simulink model "udp_scenario"  (R2024b)
settings: Solver=FixedStepDiscrete  StartTime=0.0  StopTime=90  RelTol=1e-3
model workspace (MAT data in the model file):
  firstWarning = 1
  originalScenarioChecksum = 'E10BFE42C1659D1EFEE8B4DF190BE309'
libraries: drivingscenarioandsensors x1
settings Model: Creator=jheitmann  LastModifiedBy=jheitmann

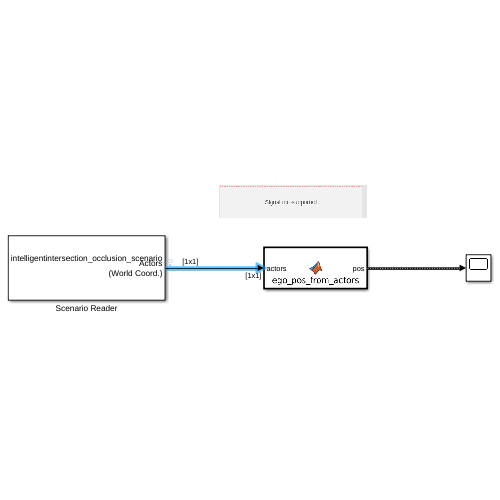
[thumbnail: Simulink's stored preview of the top-level diagram]
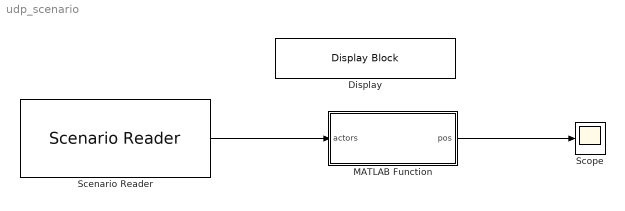
== system udp_scenario ==
  Display : DisplayBlock  LabelPosition=Hide  Transparency=1
  MATLAB Function : MATLAB Function  TreatAsAtomicUnit=on
  Scenario Reader : drivingscenarioandsensors/Scenario Reader  ScenarioSource=From file  ScenarioFileName=/home/jheitmann/MATLAB/Projects/intintersection/intelligentintersection_occlusion_scenario.mat  ScenarioVariableName=scenario  OutputCoordinateSystem=World coordinates  EgoVehicleSource=Scenario  EgoVehicleActorID=2  OrientVehiclesOnRoad=off  OutputEgoVehiclePose=on  OutputEgoVehicleState=on  SampleTime=0.1  LaneBoundaryOutput=None  LaneBoundaryDistance=0:0.5:9.5  LaneBoundaryLocation=Center of lane markings  BusNameSource=Auto  BusName=BusActors  BusNumActorsSource=Scenario  BusNumActors=100  BusName2Source=Auto  BusName2=BusLaneBoundaries  BusNumLaneBoundariesSource=Scenario  BusNumLaneBoundaries=10  BusName3Source=Auto  BusName3=BusEgoActor  BusName4Source=Auto  BusName4=BusEgoState  ShowCoordinateLabels=on  SimulateUsing=Interpreted execution
  Scope : Scope
  wires:
  MATLAB Function/1(pos) -> Scope/1
  Scenario Reader/1 -> MATLAB Function/1(actors)

== matlab function udp_scenario/MATLAB Function ==
  data: actors input; pos output
function pos = ego_pos_from_actors(actors)


pos = actors
